simulink model "NanoBalancer_Encoder"  (R2026b)
settings: Solver=daessc  StopTime=4  MaxStep=1e-4  RelTol=1e-4
PreLoadFcn:
  | InitNanoBalancer
InitFcn:
  | InitNanoBalancer
values from neighbouring files (symbols this model uses):
  bump_dt = 0.02    [check_predictor.m]    (also in run_NanoBalancer_Encoder.m; run_NanoBalancer_Stabilizer.m)
  bump_t = 1    [check_predictor.m]    (also in run_NanoBalancer_Encoder.m; run_NanoBalancer_Stabilizer.m)
  enc_a = NB.Ts/(NB.Ts + enc_tau)    [InitNanoBalancer.m]
  EncoderMode = runs{k,3}    [run_NanoBalancer_Encoder.m]
  FrictionComp = 1    [run_NanoBalancer_Encoder.m]
  KF_Ad = NB.Ad    [InitNanoBalancer.m]
  KF_Bd = NB.Bd    [InitNanoBalancer.m]
  KF_ff = [FrictionComp*NB.R*0.08, NB.r]    [InitNanoBalancer.m]
  KF_L = Pm*KF_C.'/(KF_C*Pm*KF_C.' + KF_R)    [InitNanoBalancer.m]
  sampleTime = NB.Ts    [InitNanoBalancer.m]
  SensorMode = m; InitNanoBalancer    [check_predictor.m]    (also in run_NanoBalancer_Encoder.m = runs{k,2}; run_NanoBalancer_Stabilizer.m)
  x0 = [deg2rad(theta0_deg); 0; 0; 0]    [InitNanoBalancer.m]
undefined symbols (not defined in the file or in its folder): GM, NB
libraries: fl_lib x20, nesl_utility x14, simulink x4, ee_lib x4, sdl_lib x2, sl_discontinuities x2
settings Model: Creator=arkad  LastModifiedBy=arkad
settings SimscapeCC: SimscapeLogType=all  SimscapeNominalValues="[{\"value\":\"1\",\"unit\":\"A\"},{\"value\":\"1\",\"unit\":\"bar\"},{\"value\":\"1\",\"unit\":\"cm^2\"},{\"value\":\"1\",\"unit\":\"cm^3/s\"},{\"value\":\"1\",\"unit\":\"kJ/kg\"},{\"value\":\"1\",\"unit\":\"kW\"},{\"value\":\"1\",\"unit\":\"l\"},{\"value\":\"1\",\"unit\":\"N\"},{\"value\":\"1\",\"unit\":\"N*m\"},{\"value\":\"1\",\"unit\":\"V\"},{\"value\":\"0.001\",\"unit\":\"Wb\"}]"  SimscapeUseEnergyAccounting=off

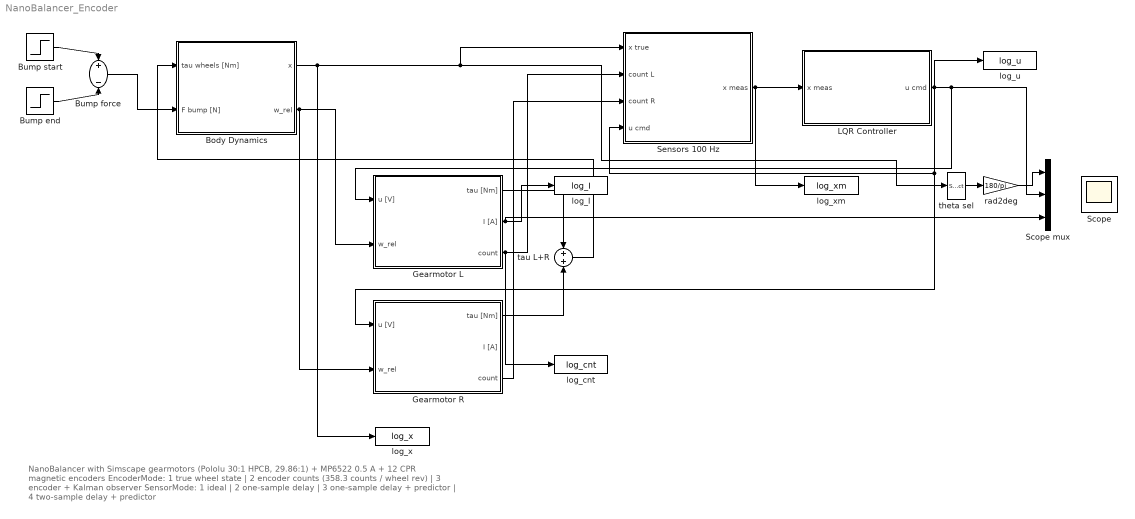
== system NanoBalancer_Encoder ==
  note: NanoBalancer with Simscape gearmotors (Pololu 30:1 HPCB, 29.86:1) + MP6522 0.5 A + 12 CPR magnetic encoders
      | EncoderMode: 1 true wheel state | 2 encoder counts (358.3 counts / wheel rev) | 3 encoder + Kalman observer
      | SensorMode: 1 ideal | 2 one-sample delay | 3 one-sample delay + predictor | 4 two-sample delay + predictor
  Body Dynamics : Subsystem
  Bump end : Step  Time=bump_t+bump_dt  FinalValue=bump_F  SampleTime=0
  Bump force : Sum  Inputs=+-
  Bump start : Step  Time=bump_t  FinalValue=bump_F  SampleTime=0
  Gearmotor L : Subsystem
  Gearmotor R : Subsystem
  LQR Controller : Subsystem
  Scope : Scope
  Scope mux : Mux  Inputs=3
  Sensors 100 Hz : Subsystem
  log_I : ToWorkspace  VariableName=log_I  SaveFormat=Structure With Time  SampleTime=-1
  log_cnt : ToWorkspace  VariableName=log_cnt  SaveFormat=Structure With Time  SampleTime=-1
  log_u : ToWorkspace  VariableName=log_u  SaveFormat=Structure With Time  SampleTime=-1
  log_x : ToWorkspace  VariableName=log_x  SaveFormat=Structure With Time  SampleTime=-1
  log_xm : ToWorkspace  VariableName=log_xm  SaveFormat=Structure With Time  SampleTime=-1
  rad2deg : Gain  Gain=180/pi
  tau L+R : Sum
  theta sel : Selector  InputPortWidth=4  IndexOptions=Index vector (dialog)  Indices=1  OutputSizes=1
  wires:
  Bump start/1 -> Bump force/1
  Bump end/1 -> Bump force/2
  Body Dynamics/2(w_rel) -> Gearmotor L/2(w_rel), Gearmotor R/2(w_rel)
  Gearmotor L/1(tau [Nm]) -> tau L+R/1
  Gearmotor R/1(tau [Nm]) -> tau L+R/2
  tau L+R/1 -> Body Dynamics/1(tau wheels [Nm])
  Bump force/1 -> Body Dynamics/2(F bump [N])
  Body Dynamics/1(x) -> theta sel/1, Sensors 100 Hz/1(x true), log_x/1
  Gearmotor L/3(count) -> Sensors 100 Hz/2(count L), log_cnt/1
  Gearmotor R/3(count) -> Sensors 100 Hz/3(count R)
  Sensors 100 Hz/1(x meas) -> LQR Controller/1(x meas), log_xm/1
  LQR Controller/1(u cmd) -> Gearmotor L/1(u [V]), Scope mux/2, Gearmotor R/1(u [V]), Sensors 100 Hz/4(u cmd), log_u/1
  Gearmotor L/2(I [A]) -> log_I/1, Scope mux/3
  theta sel/1 -> rad2deg/1
  rad2deg/1 -> Scope mux/1

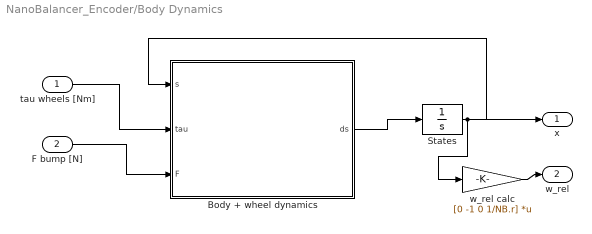
== system NanoBalancer_Encoder/Body Dynamics ==
  tau wheels [Nm] : Inport
  F bump [N] : Inport  Port=2
  Body + wheel dynamics : MATLAB Function  TreatAsAtomicUnit=on
  States : Integrator  InitialCondition=x0
  w_rel calc : Gain  Gain=[0 -1 0 1/NB.r]  Multiplication=Matrix(K*u)
  x : Outport
  w_rel : Outport  Port=2
  wires:
  States/1 -> Body + wheel dynamics/1(s), x/1, w_rel calc/1
  tau wheels [Nm]/1 -> Body + wheel dynamics/2(tau)
  F bump [N]/1 -> Body + wheel dynamics/3(F)
  Body + wheel dynamics/1(ds) -> States/1
  w_rel calc/1 -> w_rel/1

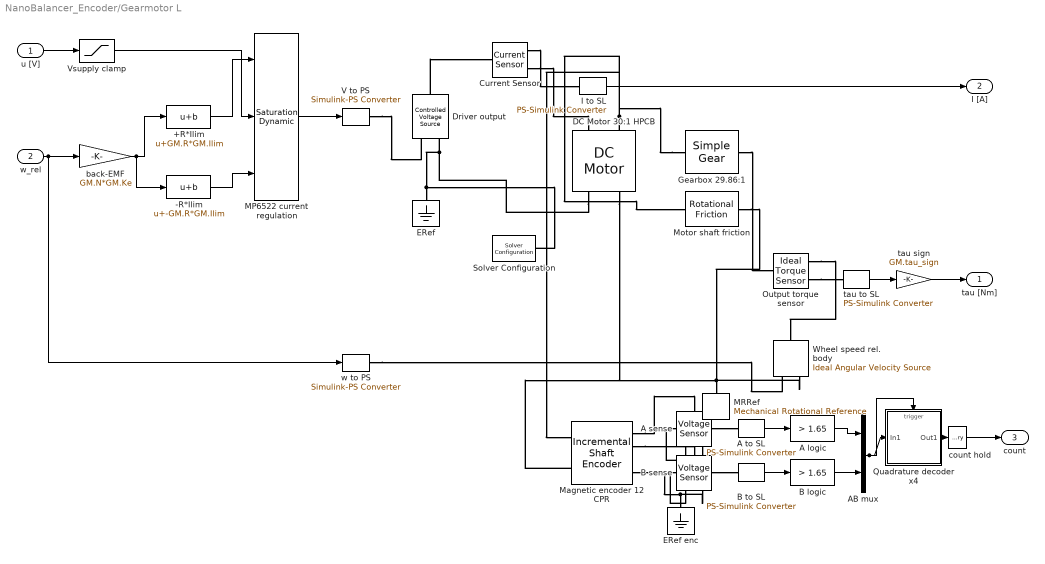
== system NanoBalancer_Encoder/Gearmotor L ==
  u [V] : Inport
  w_rel : Inport  Port=2
  +R*Ilim : Bias  Bias=GM.R*GM.Ilim  SaturateOnIntegerOverflow=off
  -R*Ilim : Bias  Bias=-GM.R*GM.Ilim  SaturateOnIntegerOverflow=off
  A logic : simulink/Logic and Bit Operations/Compare To Constant  relop=>  const=1.65  OutDataTypeStr=boolean
  A sense : fl_lib/Electrical/Electrical Sensors/Voltage Sensor
  A to SL : nesl_utility/PS-Simulink Converter  PhysicalDomain=network_engine_domain  SubClassName=ps_output  LeftPortType=input  RightPortType=output  PseudoPeriodic=off  Frequencies=[]  VectorFormat=inherit  Unit=inherit  AffineConversion=off
  AB mux : Mux  Inputs=2
  B logic : simulink/Logic and Bit Operations/Compare To Constant  relop=>  const=1.65  OutDataTypeStr=boolean
  B sense : fl_lib/Electrical/Electrical Sensors/Voltage Sensor
  B to SL : nesl_utility/PS-Simulink Converter  PhysicalDomain=network_engine_domain  SubClassName=ps_output  LeftPortType=input  RightPortType=output  PseudoPeriodic=off  Frequencies=[]  VectorFormat=inherit  Unit=inherit  AffineConversion=off
  Current Sensor : fl_lib/Electrical/Electrical Sensors/Current Sensor
  DC Motor 30:1 HPCB : ee_lib/Electromechanical/Brushed Motors/DC Motor  field_option=ee.enum.field_option.pm  Rf=100 Ohm  Lf=1 H  Laf=0.15 H  If0=0 A  parameterization=ee.enum.dcparam_option.circuit_param  Ra=GM.R Ohm  La=GM.La H  emf_or_torque=ee.enum.emf_or_torque.kv  Kv=GM.Ke V/(rad/s)  Ki=6.876e-4 N*m/A  T_stall=0.24e-3 N*m  w_max=19100 rpm  w_rated=15000 rpm  P_rated=0.08 W  V_rated=1.5 V  lam_param=ee.enum.lam_param.damping  i_noload=0 A  V_i_noload=1.5 V  J=GM.J_rotor kg*m^2  lam=0 N*m*s/rad  speed0=0 rpm  alpha=3.93e-3 1/K  Tmeas=25 degC  thermal_mass=100 J/K  initial_temperature=25 degC
  Driver output : fl_lib/Electrical/Electrical Sources/Controlled Voltage Source
  ERef : fl_lib/Electrical/Electrical Elements/Electrical Reference
  ERef enc : fl_lib/Electrical/Electrical Elements/Electrical Reference
  Gearbox 29.86:1 : sdl_lib/Gears/Simple Gear  ratio=GM.N  rotation_direction=1  friction_model=sdl.enum.gear_efficiencies_load.constant  T_noload=0.1 N*m  T_nom=5 N*m  efficiency_nom=0.8  efficiency=GM.eta_gb  temperature_TLU=[280, 300, 320] K  load_TLU=[1, 5, 10] N*m  efficiency_TLU=[.95, .9, .85]  efficiency_TLU2=[.85, .8, .75; .95, .9, .85; .85, .8, .7]  w_thr=0.5 rad/s  pwr_thr=0.001 W  enable_backlash=false  hardstop_model=simscape.enum.hardstop.smooth  backlash_distance=1e-3 mm  r_base=0.1 m  transition=1e-4 mm  backlash_stiffness=1e6 N/m  backlash_damping=1e3 N*s/m  coeff_rest=0.7  v_tol=0.001 m/s  f_tol=0.001 N  tau=0.1 s  mu_visc=[0, 0] N*m*s/rad  thermal_mass=50 J/K  temperature_specify=off  temperature_priority=High  temperature=300 K  temperature_nominal_specify=off  temperature_nominal_value=1  temperature_nominal_unit=K  x_backlash_specify=off  x_backlash_priority=None  x_backlash=0 mm  x_backlash_nominal_specify=off  x_backlash_nominal_value=1  x_backlash_nominal_unit=mm  f_hardstop_specify=off  f_hardstop_priority=None  f_hardstop=0 N  f_hardstop_nominal_specify=off  f_hardstop_nominal_value=1  f_hardstop_nominal_unit=N  v_backlash_specify=off  v_backlash_priority=None  v_backlash=0 m/s  v_backlash_nominal_specify=off  v_backlash_nominal_value=1  v_backlash_nominal_unit=m/s
  I to SL : nesl_utility/PS-Simulink Converter  PhysicalDomain=network_engine_domain  SubClassName=ps_output  LeftPortType=input  RightPortType=output  PseudoPeriodic=off  Frequencies=[]  VectorFormat=inherit  Unit=inherit  AffineConversion=off
  MP6522 current regulation : sl_discontinuities/Saturation Dynamic  OutMin=[]  OutMax=[]  OutDataTypeStr=Inherit: Same as second input  OutDataType=fixdt(1, 16)  OutScaling=2^-10  DoSatur=off
      settings: LibrarySourceBlock=|
      | simulink/Discontinuities/Saturation
      | Dynamic
  MRRef : fl_lib/Mechanical/Rotational Elements/Mechanical Rotational Reference
  Magnetic encoder 12 CPR : ee_lib/Sensors & Transducers/Incremental Shaft Encoder  NPulse=GM.PPR  Vm=3.3 V  angle0=1 deg
  Motor shaft friction : fl_lib/Mechanical/Rotational Elements/Rotational Friction  brkwy_trq=GM.Tc N*m  brkwy_vel=1 rad/s  Col_trq=GM.Tc N*m  visc_coef=0 N*m*s/rad  w_specify=off  w_priority=None  w=0 rad/s  w_nominal_specify=off  w_nominal_value=1  w_nominal_unit=rad/s  t_specify=off  t_priority=None  t=0 N*m  t_nominal_specify=off  t_nominal_value=1  t_nominal_unit=N*m
  Output torque sensor : fl_lib/Mechanical/Mechanical Sensors/Ideal Torque Sensor
  Quadrature decoder x4 : Subsystem  TreatAsAtomicUnit=on
  Solver Configuration : nesl_utility/Solver Configuration  PhysicalDomain=network_engine_domain  SubClassName=solver  LeftPortType=input  RightPortType=generic  Tones=[]  Harmonics=[]  SimulateNoise=off  Profile=off  UseLocalSampling=off  EnableSwitchedLinearOptims=on  FrequencyDomain=off  UseCCode=off  RelTol=0.001  AbsTol=0.001  MinStep=1e-09  ToWorkspace=off  RevertToSquareIcSolve=off  NumHomotopyIterations=100  PhasorMode=off  PhasorModeNumHarmonics=1  ConsistencySolver=NEWTON_XTOL_AFTER_FTOL  CanonicalOrdering=CANONICAL  OptimizeIntermediates=OPTIMIZED  MulticoreSolverChoice=BACKWARD_EULER  IndexReductionMethod=DerivativeReplacement  DoDC=off  ResidualTolerance=1e-09  ConsistencyTolSource=GLOBAL  ConsistencyAbsTol=0.001  ConsistencyRelTol=0.001  ConsistencyTolFactor=0.001  UseLocalSolver=off  LocalSolverChoice=NE_BACKWARD_EULER_ADVANCER  ResolveIndetEquations=on  FunctionEvalNumThread=1  LocalSolverSampleTime=0.001  DoFixedCost=off  MaxNonlinIter=3  MaxModeIter=2  ComputeImpulses=off  ImpulseIterations=2  LinearAlgebra=auto  LinearAlgebraNumThread=0  EquationFormulation=NE_TIME_EF  DelaysMemoryBudget=1024  AutomaticFiltering=on  FilteringTimeConstant=0.001  PartitionStorageMethod=AS_NEEDED  PartitionMemoryBudget=1024  PartitionMethod=BALANCED  MultibodyUseLocalSolver=off  MultibodyLocalSolverChoice=ODE1  MultibodyLocalSolverSampleTime=0.001
  V to PS : nesl_utility/Simulink-PS Converter  PhysicalDomain=network_engine_domain  SubClassName=ps_input  LeftPortType=input  RightPortType=output  PseudoPeriodic=off  Frequencies=[]  NoiseDistribution=none  NoiseParameters=[]  Unit=1  AffineConversion=off  FilteringAndDerivatives=provide  SimscapeFilterOrder=1  InputFilterTimeConstant=0.001  UdotUserProvided=0
  Vsupply clamp : Saturate  UpperLimit=GM.Vmax  LowerLimit=-GM.Vmax
  Wheel speed rel. body : fl_lib/Mechanical/Mechanical Sources/Ideal Angular Velocity Source
  back-EMF : Gain  Gain=GM.N*GM.Ke
  count hold : Memory
  tau sign : Gain  Gain=GM.tau_sign
  tau to SL : nesl_utility/PS-Simulink Converter  PhysicalDomain=network_engine_domain  SubClassName=ps_output  LeftPortType=input  RightPortType=output  PseudoPeriodic=off  Frequencies=[]  VectorFormat=inherit  Unit=inherit  AffineConversion=off
  w to PS : nesl_utility/Simulink-PS Converter  PhysicalDomain=network_engine_domain  SubClassName=ps_input  LeftPortType=input  RightPortType=output  PseudoPeriodic=off  Frequencies=[]  NoiseDistribution=none  NoiseParameters=[]  Unit=1  AffineConversion=off  FilteringAndDerivatives=filter  SimscapeFilterOrder=2  InputFilterTimeConstant=2e-4  UdotUserProvided=0
  tau [Nm] : Outport
  I [A] : Outport  Port=2
  count : Outport  Port=3
  wires:
  u [V]/1 -> Vsupply clamp/1
  w_rel/1 -> back-EMF/1, w to PS/1
  back-EMF/1 -> +R*Ilim/1, -R*Ilim/1
  +R*Ilim/1 -> MP6522 current regulation/1
  Vsupply clamp/1 -> MP6522 current regulation/2
  -R*Ilim/1 -> MP6522 current regulation/3
  MP6522 current regulation/1 -> V to PS/1
  tau to SL/1 -> tau sign/1
  tau sign/1 -> tau [Nm]/1
  I to SL/1 -> I [A]/1
  A to SL/1 -> A logic/1
  B to SL/1 -> B logic/1
  A logic/1 -> AB mux/1
  B logic/1 -> AB mux/2
  AB mux/1 -> Quadrature decoder x4/1(In1), Quadrature decoder x4/Trigger
  Quadrature decoder x4/1(Out1) -> count hold/1
  count hold/1 -> count/1
  connections:
  V to PS/RConn1 -- Driver output/RConn1
  Driver output/LConn1 -- Current Sensor/LConn1
  Current Sensor/RConn2 -- DC Motor 30:1 HPCB/LConn1
  Current Sensor/RConn1 -- I to SL/LConn1
  Driver output/RConn2 -- DC Motor 30:1 HPCB/RConn1 -- ERef/LConn1 -- Solver Configuration/RConn1
  Gearbox 29.86:1/LConn1 -- DC Motor 30:1 HPCB/LConn2 -- Motor shaft friction/LConn1 -- Magnetic encoder 12 CPR/LConn1
  Motor shaft friction/RConn1 -- DC Motor 30:1 HPCB/RConn2 -- Wheel speed rel. body/RConn2 -- MRRef/LConn1 -- Magnetic encoder 12 CPR/LConn2
  Gearbox 29.86:1/RConn1 -- Output torque sensor/LConn1
  Output torque sensor/RConn1 -- Wheel speed rel. body/LConn1
  w to PS/RConn1 -- Wheel speed rel. body/RConn1
  Output torque sensor/RConn2 -- tau to SL/LConn1
  Magnetic encoder 12 CPR/RConn4 -- A sense/RConn2 -- ERef enc/LConn1 -- B sense/RConn2
  Magnetic encoder 12 CPR/RConn1 -- A sense/LConn1
  Magnetic encoder 12 CPR/RConn2 -- B sense/LConn1
  A sense/RConn1 -- A to SL/LConn1
  B sense/RConn1 -- B to SL/LConn1

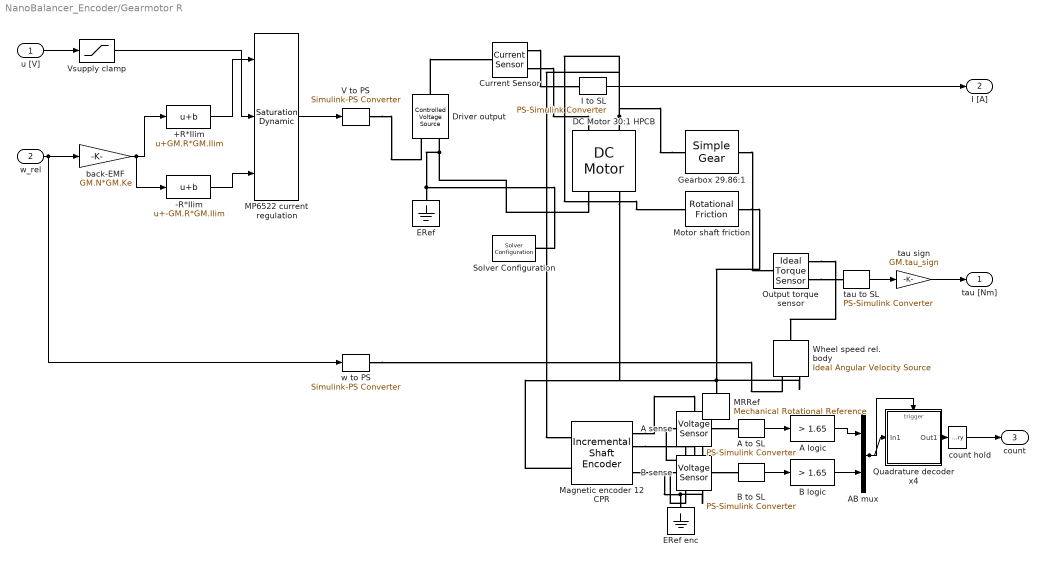
== system NanoBalancer_Encoder/Gearmotor R ==
  u [V] : Inport
  w_rel : Inport  Port=2
  +R*Ilim : Bias  Bias=GM.R*GM.Ilim  SaturateOnIntegerOverflow=off
  -R*Ilim : Bias  Bias=-GM.R*GM.Ilim  SaturateOnIntegerOverflow=off
  A logic : simulink/Logic and Bit Operations/Compare To Constant  relop=>  const=1.65  OutDataTypeStr=boolean
  A sense : fl_lib/Electrical/Electrical Sensors/Voltage Sensor
  A to SL : nesl_utility/PS-Simulink Converter  PhysicalDomain=network_engine_domain  SubClassName=ps_output  LeftPortType=input  RightPortType=output  PseudoPeriodic=off  Frequencies=[]  VectorFormat=inherit  Unit=inherit  AffineConversion=off
  AB mux : Mux  Inputs=2
  B logic : simulink/Logic and Bit Operations/Compare To Constant  relop=>  const=1.65  OutDataTypeStr=boolean
  B sense : fl_lib/Electrical/Electrical Sensors/Voltage Sensor
  B to SL : nesl_utility/PS-Simulink Converter  PhysicalDomain=network_engine_domain  SubClassName=ps_output  LeftPortType=input  RightPortType=output  PseudoPeriodic=off  Frequencies=[]  VectorFormat=inherit  Unit=inherit  AffineConversion=off
  Current Sensor : fl_lib/Electrical/Electrical Sensors/Current Sensor
  DC Motor 30:1 HPCB : ee_lib/Electromechanical/Brushed Motors/DC Motor  field_option=ee.enum.field_option.pm  Rf=100 Ohm  Lf=1 H  Laf=0.15 H  If0=0 A  parameterization=ee.enum.dcparam_option.circuit_param  Ra=GM.R Ohm  La=GM.La H  emf_or_torque=ee.enum.emf_or_torque.kv  Kv=GM.Ke V/(rad/s)  Ki=6.876e-4 N*m/A  T_stall=0.24e-3 N*m  w_max=19100 rpm  w_rated=15000 rpm  P_rated=0.08 W  V_rated=1.5 V  lam_param=ee.enum.lam_param.damping  i_noload=0 A  V_i_noload=1.5 V  J=GM.J_rotor kg*m^2  lam=0 N*m*s/rad  speed0=0 rpm  alpha=3.93e-3 1/K  Tmeas=25 degC  thermal_mass=100 J/K  initial_temperature=25 degC
  Driver output : fl_lib/Electrical/Electrical Sources/Controlled Voltage Source
  ERef : fl_lib/Electrical/Electrical Elements/Electrical Reference
  ERef enc : fl_lib/Electrical/Electrical Elements/Electrical Reference
  Gearbox 29.86:1 : sdl_lib/Gears/Simple Gear  ratio=GM.N  rotation_direction=1  friction_model=sdl.enum.gear_efficiencies_load.constant  T_noload=0.1 N*m  T_nom=5 N*m  efficiency_nom=0.8  efficiency=GM.eta_gb  temperature_TLU=[280, 300, 320] K  load_TLU=[1, 5, 10] N*m  efficiency_TLU=[.95, .9, .85]  efficiency_TLU2=[.85, .8, .75; .95, .9, .85; .85, .8, .7]  w_thr=0.5 rad/s  pwr_thr=0.001 W  enable_backlash=false  hardstop_model=simscape.enum.hardstop.smooth  backlash_distance=1e-3 mm  r_base=0.1 m  transition=1e-4 mm  backlash_stiffness=1e6 N/m  backlash_damping=1e3 N*s/m  coeff_rest=0.7  v_tol=0.001 m/s  f_tol=0.001 N  tau=0.1 s  mu_visc=[0, 0] N*m*s/rad  thermal_mass=50 J/K  temperature_specify=off  temperature_priority=High  temperature=300 K  temperature_nominal_specify=off  temperature_nominal_value=1  temperature_nominal_unit=K  x_backlash_specify=off  x_backlash_priority=None  x_backlash=0 mm  x_backlash_nominal_specify=off  x_backlash_nominal_value=1  x_backlash_nominal_unit=mm  f_hardstop_specify=off  f_hardstop_priority=None  f_hardstop=0 N  f_hardstop_nominal_specify=off  f_hardstop_nominal_value=1  f_hardstop_nominal_unit=N  v_backlash_specify=off  v_backlash_priority=None  v_backlash=0 m/s  v_backlash_nominal_specify=off  v_backlash_nominal_value=1  v_backlash_nominal_unit=m/s
  I to SL : nesl_utility/PS-Simulink Converter  PhysicalDomain=network_engine_domain  SubClassName=ps_output  LeftPortType=input  RightPortType=output  PseudoPeriodic=off  Frequencies=[]  VectorFormat=inherit  Unit=inherit  AffineConversion=off
  MP6522 current regulation : sl_discontinuities/Saturation Dynamic  OutMin=[]  OutMax=[]  OutDataTypeStr=Inherit: Same as second input  OutDataType=fixdt(1, 16)  OutScaling=2^-10  DoSatur=off
      settings: LibrarySourceBlock=|
      | simulink/Discontinuities/Saturation
      | Dynamic
  MRRef : fl_lib/Mechanical/Rotational Elements/Mechanical Rotational Reference
  Magnetic encoder 12 CPR : ee_lib/Sensors & Transducers/Incremental Shaft Encoder  NPulse=GM.PPR  Vm=3.3 V  angle0=1 deg
  Motor shaft friction : fl_lib/Mechanical/Rotational Elements/Rotational Friction  brkwy_trq=GM.Tc N*m  brkwy_vel=1 rad/s  Col_trq=GM.Tc N*m  visc_coef=0 N*m*s/rad  w_specify=off  w_priority=None  w=0 rad/s  w_nominal_specify=off  w_nominal_value=1  w_nominal_unit=rad/s  t_specify=off  t_priority=None  t=0 N*m  t_nominal_specify=off  t_nominal_value=1  t_nominal_unit=N*m
  Output torque sensor : fl_lib/Mechanical/Mechanical Sensors/Ideal Torque Sensor
  Quadrature decoder x4 : Subsystem  TreatAsAtomicUnit=on
  Solver Configuration : nesl_utility/Solver Configuration  PhysicalDomain=network_engine_domain  SubClassName=solver  LeftPortType=input  RightPortType=generic  Tones=[]  Harmonics=[]  SimulateNoise=off  Profile=off  UseLocalSampling=off  EnableSwitchedLinearOptims=on  FrequencyDomain=off  UseCCode=off  RelTol=0.001  AbsTol=0.001  MinStep=1e-09  ToWorkspace=off  RevertToSquareIcSolve=off  NumHomotopyIterations=100  PhasorMode=off  PhasorModeNumHarmonics=1  ConsistencySolver=NEWTON_XTOL_AFTER_FTOL  CanonicalOrdering=CANONICAL  OptimizeIntermediates=OPTIMIZED  MulticoreSolverChoice=BACKWARD_EULER  IndexReductionMethod=DerivativeReplacement  DoDC=off  ResidualTolerance=1e-09  ConsistencyTolSource=GLOBAL  ConsistencyAbsTol=0.001  ConsistencyRelTol=0.001  ConsistencyTolFactor=0.001  UseLocalSolver=off  LocalSolverChoice=NE_BACKWARD_EULER_ADVANCER  ResolveIndetEquations=on  FunctionEvalNumThread=1  LocalSolverSampleTime=0.001  DoFixedCost=off  MaxNonlinIter=3  MaxModeIter=2  ComputeImpulses=off  ImpulseIterations=2  LinearAlgebra=auto  LinearAlgebraNumThread=0  EquationFormulation=NE_TIME_EF  DelaysMemoryBudget=1024  AutomaticFiltering=on  FilteringTimeConstant=0.001  PartitionStorageMethod=AS_NEEDED  PartitionMemoryBudget=1024  PartitionMethod=BALANCED  MultibodyUseLocalSolver=off  MultibodyLocalSolverChoice=ODE1  MultibodyLocalSolverSampleTime=0.001
  V to PS : nesl_utility/Simulink-PS Converter  PhysicalDomain=network_engine_domain  SubClassName=ps_input  LeftPortType=input  RightPortType=output  PseudoPeriodic=off  Frequencies=[]  NoiseDistribution=none  NoiseParameters=[]  Unit=1  AffineConversion=off  FilteringAndDerivatives=provide  SimscapeFilterOrder=1  InputFilterTimeConstant=0.001  UdotUserProvided=0
  Vsupply clamp : Saturate  UpperLimit=GM.Vmax  LowerLimit=-GM.Vmax
  Wheel speed rel. body : fl_lib/Mechanical/Mechanical Sources/Ideal Angular Velocity Source
  back-EMF : Gain  Gain=GM.N*GM.Ke
  count hold : Memory
  tau sign : Gain  Gain=GM.tau_sign
  tau to SL : nesl_utility/PS-Simulink Converter  PhysicalDomain=network_engine_domain  SubClassName=ps_output  LeftPortType=input  RightPortType=output  PseudoPeriodic=off  Frequencies=[]  VectorFormat=inherit  Unit=inherit  AffineConversion=off
  w to PS : nesl_utility/Simulink-PS Converter  PhysicalDomain=network_engine_domain  SubClassName=ps_input  LeftPortType=input  RightPortType=output  PseudoPeriodic=off  Frequencies=[]  NoiseDistribution=none  NoiseParameters=[]  Unit=1  AffineConversion=off  FilteringAndDerivatives=filter  SimscapeFilterOrder=2  InputFilterTimeConstant=2e-4  UdotUserProvided=0
  tau [Nm] : Outport
  I [A] : Outport  Port=2
  count : Outport  Port=3
  wires:
  u [V]/1 -> Vsupply clamp/1
  w_rel/1 -> back-EMF/1, w to PS/1
  back-EMF/1 -> +R*Ilim/1, -R*Ilim/1
  +R*Ilim/1 -> MP6522 current regulation/1
  Vsupply clamp/1 -> MP6522 current regulation/2
  -R*Ilim/1 -> MP6522 current regulation/3
  MP6522 current regulation/1 -> V to PS/1
  tau to SL/1 -> tau sign/1
  tau sign/1 -> tau [Nm]/1
  I to SL/1 -> I [A]/1
  A to SL/1 -> A logic/1
  B to SL/1 -> B logic/1
  A logic/1 -> AB mux/1
  B logic/1 -> AB mux/2
  AB mux/1 -> Quadrature decoder x4/1(In1), Quadrature decoder x4/Trigger
  Quadrature decoder x4/1(Out1) -> count hold/1
  count hold/1 -> count/1
  connections:
  V to PS/RConn1 -- Driver output/RConn1
  Driver output/LConn1 -- Current Sensor/LConn1
  Current Sensor/RConn2 -- DC Motor 30:1 HPCB/LConn1
  Current Sensor/RConn1 -- I to SL/LConn1
  Driver output/RConn2 -- DC Motor 30:1 HPCB/RConn1 -- ERef/LConn1 -- Solver Configuration/RConn1
  Gearbox 29.86:1/LConn1 -- DC Motor 30:1 HPCB/LConn2 -- Motor shaft friction/LConn1 -- Magnetic encoder 12 CPR/LConn1
  Motor shaft friction/RConn1 -- DC Motor 30:1 HPCB/RConn2 -- Wheel speed rel. body/RConn2 -- MRRef/LConn1 -- Magnetic encoder 12 CPR/LConn2
  Gearbox 29.86:1/RConn1 -- Output torque sensor/LConn1
  Output torque sensor/RConn1 -- Wheel speed rel. body/LConn1
  w to PS/RConn1 -- Wheel speed rel. body/RConn1
  Output torque sensor/RConn2 -- tau to SL/LConn1
  Magnetic encoder 12 CPR/RConn4 -- A sense/RConn2 -- ERef enc/LConn1 -- B sense/RConn2
  Magnetic encoder 12 CPR/RConn1 -- A sense/LConn1
  Magnetic encoder 12 CPR/RConn2 -- B sense/LConn1
  A sense/RConn1 -- A to SL/LConn1
  B sense/RConn1 -- B to SL/LConn1

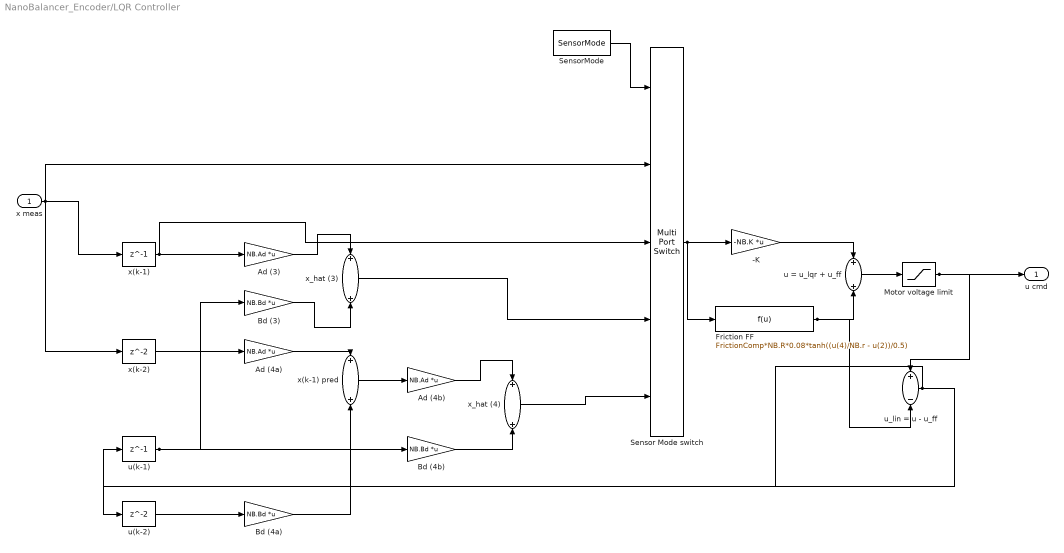
== system NanoBalancer_Encoder/LQR Controller ==
  x meas : Inport
  -K : Gain  Gain=-NB.K  Multiplication=Matrix(K*u)
  Ad (3) : Gain  Gain=NB.Ad  Multiplication=Matrix(K*u)
  Ad (4a) : Gain  Gain=NB.Ad  Multiplication=Matrix(K*u)
  Ad (4b) : Gain  Gain=NB.Ad  Multiplication=Matrix(K*u)
  Bd (3) : Gain  Gain=NB.Bd  Multiplication=Matrix(K*u)
  Bd (4a) : Gain  Gain=NB.Bd  Multiplication=Matrix(K*u)
  Bd (4b) : Gain  Gain=NB.Bd  Multiplication=Matrix(K*u)
  Friction FF : Fcn  Expr=FrictionComp*NB.R*0.08*tanh((u(4)/NB.r - u(2))/0.5)
  Motor voltage limit : Saturate  UpperLimit=NB.Vmax  LowerLimit=-NB.Vmax
  Sensor Mode switch : MultiPortSwitch  Inputs=4  SaturateOnIntegerOverflow=off  InputSameDT=off
  SensorMode : Constant  Value=SensorMode
  u = u_lqr + u_ff : Sum
  u(k-1) : Delay  DelayLength=1  InitialCondition=0  SampleTime=sampleTime
  u(k-2) : Delay  InitialCondition=0  SampleTime=sampleTime
  u_lin = u - u_ff : Sum  Inputs=+-
  x(k-1) : Delay  DelayLength=1  InitialCondition=0  SampleTime=sampleTime
  x(k-1) pred : Sum
  x(k-2) : Delay  InitialCondition=0  SampleTime=sampleTime
  x_hat (3) : Sum
  x_hat (4) : Sum
  u cmd : Outport
  wires:
  u_lin = u - u_ff/1 -> u(k-2)/1, u(k-1)/1
  Motor voltage limit/1 -> u_lin = u - u_ff/1, u cmd/1
  u = u_lqr + u_ff/1 -> Motor voltage limit/1
  Friction FF/1 -> u_lin = u - u_ff/2, u = u_lqr + u_ff/2
  -K/1 -> u = u_lqr + u_ff/1
  Sensor Mode switch/1 -> Friction FF/1, -K/1
  x_hat (4)/1 -> Sensor Mode switch/5
  x_hat (3)/1 -> Sensor Mode switch/4
  SensorMode/1 -> Sensor Mode switch/1
  Bd (4b)/1 -> x_hat (4)/2
  Ad (4b)/1 -> x_hat (4)/1
  x(k-1) pred/1 -> Ad (4b)/1
  Bd (4a)/1 -> x(k-1) pred/2
  Ad (4a)/1 -> x(k-1) pred/1
  u(k-2)/1 -> Bd (4a)/1
  x(k-2)/1 -> Ad (4a)/1
  Bd (3)/1 -> x_hat (3)/2
  Ad (3)/1 -> x_hat (3)/1
  u(k-1)/1 -> Bd (4b)/1, Bd (3)/1
  x(k-1)/1 -> Sensor Mode switch/3, Ad (3)/1
  x meas/1 -> Sensor Mode switch/2, x(k-2)/1, x(k-1)/1

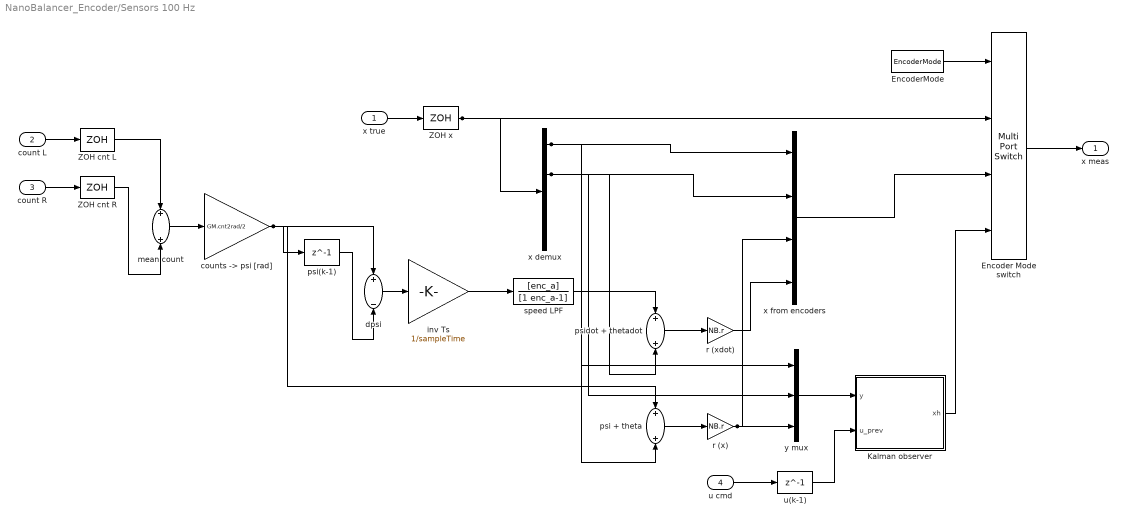
== system NanoBalancer_Encoder/Sensors 100 Hz ==
  x true : Inport
  count L : Inport  Port=2
  count R : Inport  Port=3
  u cmd : Inport  Port=4
  Encoder Mode switch : MultiPortSwitch  SaturateOnIntegerOverflow=off  InputSameDT=off
  EncoderMode : Constant  Value=EncoderMode
  Kalman observer : MATLAB Function  TreatAsAtomicUnit=on
  ZOH cnt L : ZeroOrderHold  SampleTime=sampleTime
  ZOH cnt R : ZeroOrderHold  SampleTime=sampleTime
  ZOH x : ZeroOrderHold  SampleTime=sampleTime
  "counts -> psi [rad]" : Gain  Gain=GM.cnt2rad/2
  dpsi : Sum  Inputs=+-
  inv Ts : Gain  Gain=1/sampleTime
  mean count : Sum
  psi + theta : Sum
  psi(k-1) : Delay  DelayLength=1  InitialCondition=0  SampleTime=sampleTime
  psidot + thetadot : Sum
  r (x) : Gain  Gain=NB.r
  r (xdot) : Gain  Gain=NB.r
  speed LPF : DiscreteTransferFcn  Numerator=[enc_a]  Denominator=[1 enc_a-1]  SampleTime=sampleTime
  u(k-1) : Delay  DelayLength=1  InitialCondition=0  SampleTime=sampleTime
  x demux : Demux
  x from encoders : Mux
  y mux : Mux  Inputs=3
  x meas : Outport
  wires:
  x demux/1 -> x from encoders/1, y mux/1, psi + theta/2
  psi(k-1)/1 -> dpsi/2
  "counts -> psi [rad]"/1 -> dpsi/1, psi + theta/1, psi(k-1)/1
  ZOH cnt L/1 -> mean count/1
  count L/1 -> ZOH cnt L/1
  ZOH x/1 -> Encoder Mode switch/2, x demux/1
  x true/1 -> ZOH x/1
  mean count/1 -> "counts -> psi [rad]"/1
  ZOH cnt R/1 -> mean count/2
  x demux/2 -> psidot + thetadot/2, y mux/2, x from encoders/2
  count R/1 -> ZOH cnt R/1
  dpsi/1 -> inv Ts/1
  x from encoders/1 -> Encoder Mode switch/3
  inv Ts/1 -> speed LPF/1
  Encoder Mode switch/1 -> x meas/1
  speed LPF/1 -> psidot + thetadot/1
  EncoderMode/1 -> Encoder Mode switch/1
  psidot + thetadot/1 -> r (xdot)/1
  u cmd/1 -> u(k-1)/1
  psi + theta/1 -> r (x)/1
  y mux/1 -> Kalman observer/1(y)
  r (xdot)/1 -> x from encoders/4
  r (x)/1 -> y mux/3, x from encoders/3
  u(k-1)/1 -> Kalman observer/2(u_prev)
  Kalman observer/1(xh) -> Encoder Mode switch/4

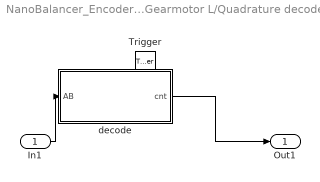
== system NanoBalancer_Encoder/Gearmotor L/Quadrature decoder x4 ==
  In1 : Inport
  Trigger : TriggerPort  TriggerType=either  VariantControl=(inherit)
  decode : MATLAB Function  TreatAsAtomicUnit=on
  Out1 : Outport  InitialOutput=0
  wires:
  In1/1 -> decode/1(AB)
  decode/1(cnt) -> Out1/1

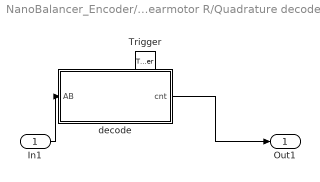
== system NanoBalancer_Encoder/Gearmotor R/Quadrature decoder x4 ==
  In1 : Inport
  Trigger : TriggerPort  TriggerType=either  VariantControl=(inherit)
  decode : MATLAB Function  TreatAsAtomicUnit=on
  Out1 : Outport  InitialOutput=0
  wires:
  In1/1 -> decode/1(AB)
  decode/1(cnt) -> Out1/1

== matlab function NanoBalancer_Encoder/Gearmotor L/Quadrature decoder x4/decode ==
  data: AB input size=[2 1]; cnt output
function cnt = decode(AB)
% x4 quadrature decoding: +1 per edge when A leads B (positive rotation)
persistent prev c
if isempty(prev), prev = 2*double(AB(1)) + double(AB(2)); c = 0; end
s = 2*double(AB(1)) + double(AB(2));
T = [0 -1 1 0; 1 0 0 -1; -1 0 0 1; 0 1 -1 0];
c = c + T(prev+1, s+1);
prev = s;
cnt = c;

== matlab function NanoBalancer_Encoder/Body Dynamics/Body + wheel dynamics ==
  data: s input size=[4 1]; ds output; tau input; F input; NB_pb parameter size=[1 7]
function ds = fcn(s, tau, F, NB_pb)
% Wheeled inverted pendulum, body + wheels only (motor rotor inertia, friction
% and torque come from the Simscape gearmotors). tau = total torque on wheels.
m_b=NB_pb(1); m_w=NB_pb(2); l=NB_pb(3); Ib=NB_pb(4); Iw=NB_pb(5); r=NB_pb(6); g=NB_pb(7);
th = s(1); thd = s(2); xd = s(4);
a = Ib + m_b*l^2;  b = m_b*r*l;  c = Iw + (m_b + m_w)*r^2;
M = [a, b*cos(th); b*cos(th), c];
f = [m_b*g*l*sin(th) - tau + F*l*cos(th); tau + b*sin(th)*thd^2 + F*r];
acc = M\f;
ds = [thd; acc(1); xd; r*acc(2)];

== matlab function NanoBalancer_Encoder/Gearmotor R/Quadrature decoder x4/decode ==
  data: AB input size=[2 1]; cnt output
function cnt = decode(AB)
% x4 quadrature decoding: +1 per edge when A leads B (positive rotation)
persistent prev c
if isempty(prev), prev = 2*double(AB(1)) + double(AB(2)); c = 0; end
s = 2*double(AB(1)) + double(AB(2));
T = [0 -1 1 0; 1 0 0 -1; -1 0 0 1; 0 1 -1 0];
c = c + T(prev+1, s+1);
prev = s;
cnt = c;

== matlab function NanoBalancer_Encoder/Sensors 100 Hz/Kalman observer ==
  data: y input size=[3 1]; xh output; u_prev input; KF_Ad parameter; KF_Bd parameter; KF_L parameter; KF_ff parameter
function xh = kf(y, u_prev, KF_Ad, KF_Bd, KF_L, KF_ff)
% Steady-state Kalman observer (current estimator), runs at the 100 Hz loop rate.
% y = [theta; theta_dot; x_enc]. Predict with the linear model and the linear
% part of the applied voltage (friction feed-forward removed), then correct.
persistent x
if isempty(x), x = zeros(4,1); end
u_lin = u_prev - KF_ff(1)*tanh((x(4)/KF_ff(2) - x(2))/0.5);
xp = KF_Ad*x + KF_Bd*u_lin;
C = [1 0 0 0; 0 1 0 0; 0 0 1 0];
x = xp + KF_L*(y - C*xp);
xh = x;
